simulink model "PMSM_SMO_Luenberger"  (R2024b)
settings: Solver=FixedStepDiscrete  StartTime=0.0  StopTime=2.4  FixedStep=TsPlant  RelTol=1e-3
InitFcn:
  | demoModel=bdroot; demoWorkspace=get_param(demoModel,'ModelWorkspace');
  | demoCases=getVariable(demoWorkspace,'DemoCases');
  | demoCaseName=get_param([demoModel '/Experiment_Settings'],'CaseName');
  | demoSelected=find(strcmp(demoCaseName,{demoCases.name}),1);
  | demoValues=demoCases(demoSelected).variables; demoNames=fieldnames(demoValues);
  | for demoIndex=1:numel(demoNames), assignin(demoWorkspace,demoNames{demoIndex},demoValues.(demoNames{demoIndex})); end
  | clear demoModel demoWorkspace demoCases demoCaseName demoSelected demoValues demoNames demoIndex;
model workspace (MAT data in the model file):
  CurrentKi = 720
  CurrentKp = 5.4
  DemoCases : object (value not decoded)
  EFilterA = 0.950976923294
  EFilterHz = 160
  FluxPM = 0.045
  FrictionB = 0.0001
  InertiaJ = 0.00025
  LsActual = 0.003
  LsNom = 0.003
  LuenL1 = 528.165269456
  LuenL2 = 575.388341705
  LuenPLLKi = 394784.176044
  LuenPLLKp = 1095.31763963
  PLLKi = 15791.3670417
  PLLKp = 177.688480487
  PWMfreq = 20000
  PolePairs = 4
  RsActual = 0.4
  RsNom = 0.4
  SmoK = 17.2906443411
  SmoKe = 0.821531981197
  SmoM = 33333.3333333
  SmoPLLKi = 116919.038546
  SmoPLLKp = 483.495044434
  SmoPhi = 0.315914362573
  SmoWmin = 100
  SpeedFilterA = 0.987512256524
  SpeedKi = 0.4
  SpeedKp = 0.04
  ThetaInitial = 0
  TsControl = 5e-05
  TsPlant = 2.5e-06
  TsSpeed = 0.001
  Vdc = 48
  inverterMode = 0
  loadStep = 0.18
  noiseTsABC = timeseries
  noiseTsABC.Name = 'unnamed'
  noiseTsABC.DataInfo = tsdata.datametadata
  noiseTsABC.DataInfo.Interpolation = tsdata.interpolation
  noiseTsABC.DataInfo.Interpolation.Fhandle : function handle (value not decoded)
  noiseTsABC.DataInfo.Interpolation.Name = 'linear'
  noiseTsABC.TimeInfo = tsdata.timemetadata
  noiseTsABC.TimeInfo.Length = 48001
  noiseTsABC.TimeInfo.DuplicateTimes = 0
  noiseTsABC.TimeInfo.Time_ = [0 5e-05 0.0001 0.00015 0.0002 0.00025 0.0003 0.00035 0.0004 0.00045 0.0005 0.00055 ... (48001 elements, 48001x1)]
  noiseTsABC.TimeInfo.Initialized = 1
  noiseTsABC.QualityInfo = tsdata.qualmetadata
  noiseTsABC.Data_ = [-0.0189584791563 -0.0055660672953 -0.00857497820907 -0.0128644236526 0.0199755803207 -0.0011001642805 0.0163280309249 -0.016225075147 0.00870875726314 -0.0018724684667 0.00550338350148 -0.000938030229996 ... (144003 elements, 48001x3)]
  rpm0 = 700
  rpm1 = 1000
  voltageErrorTs = timeseries
  voltageErrorTs.Name = 'unnamed'
  voltageErrorTs.DataInfo = tsdata.datametadata
  voltageErrorTs.DataInfo.Interpolation = tsdata.interpolation
  voltageErrorTs.DataInfo.Interpolation.Fhandle : function handle (value not decoded)
  voltageErrorTs.DataInfo.Interpolation.Name = 'linear'
  voltageErrorTs.TimeInfo = tsdata.timemetadata
  voltageErrorTs.TimeInfo.Length = 48001
  voltageErrorTs.TimeInfo.DuplicateTimes = 0
  voltageErrorTs.TimeInfo.Time_ = [0 5e-05 0.0001 0.00015 0.0002 0.00025 0.0003 0.00035 0.0004 0.00045 0.0005 0.00055 ... (48001 elements, 48001x1)]
  voltageErrorTs.TimeInfo.Initialized = 1
  voltageErrorTs.QualityInfo = tsdata.qualmetadata
  voltageErrorTs.Data_ = [0 0 0 0 0 0 0 0 0 0 0 0 ... (96002 elements, 48001x2)]
undefined symbols (not defined in the file): DiscIntNeverNeededParam
settings Model: Creator=lxy  LastModifiedBy=lxy

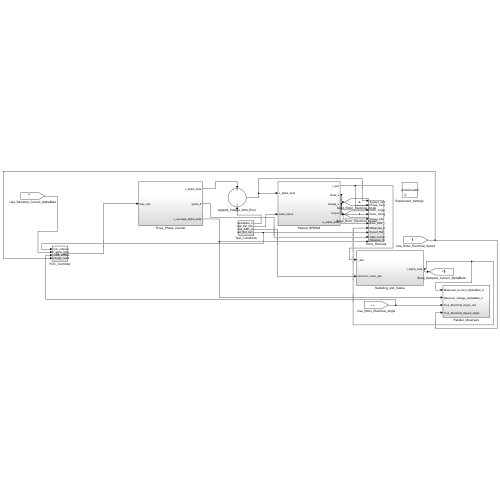
[thumbnail: Simulink's stored preview of the top-level diagram]
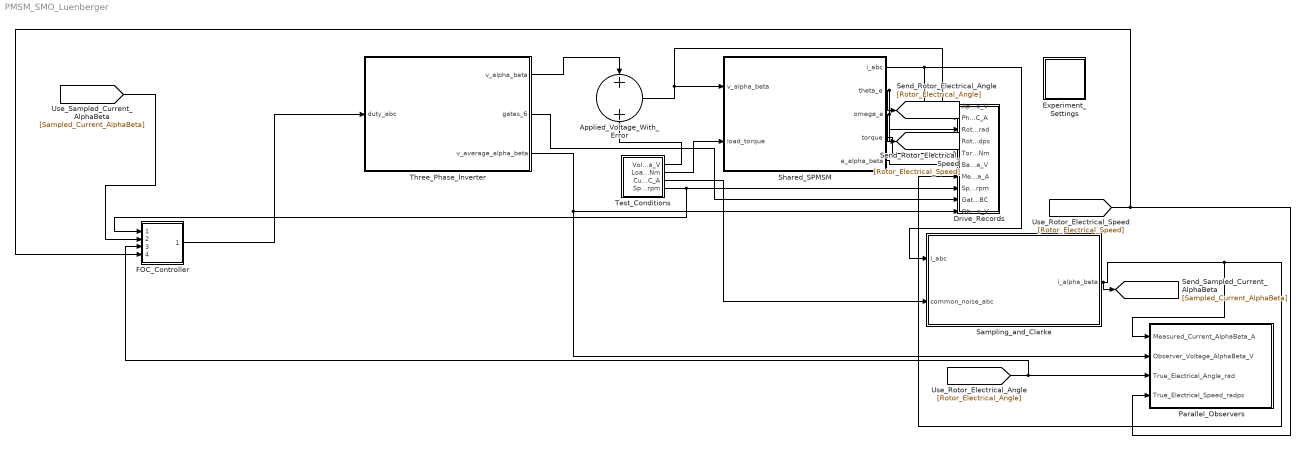
== system PMSM_SMO_Luenberger ==
  Applied_Voltage_With_Error : Sum
  Drive_Records : Subsystem
  Experiment_Settings : Subsystem  mask{CaseName=nominal}
      mask prompts: CaseName "Experiment"
      mask help: Select the experiment, then click Run. Parameters and test inputs are included in the download.
      mask TypeOptions CaseName: nominal | noise | mismatch | low_speed | zero_speed | ccf_narrow | ccf_wide | switched | voltage_bias | current_impulse | warm_resistance | heavy_load
      mask Display: disp('Experiment settings')
  FOC_Controller : Subsystem
  Parallel_Observers : Subsystem
  Sampling_and_Clarke : Subsystem
  Shared_SPMSM : Subsystem
  Test_Conditions : Subsystem
  Three_Phase_Inverter : Subsystem
  wires:
  Three_Phase_Inverter/1(v_alpha_beta) -> Applied_Voltage_With_Error/1
  Test_Conditions/3(Current_Noise_ABC_A) -> Sampling_and_Clarke/2(common_noise_abc)
  Test_Conditions/2(Load_Ref_Nm) -> Shared_SPMSM/2(load_torque)
  Test_Conditions/1(Voltage_Offset_AlphaBeta_V) -> Applied_Voltage_With_Error/2
  Shared_SPMSM/2(theta_e) -> [Rotor_Electrical_Angle], Drive_Records/3(Rotor_Angle_rad)
  Shared_SPMSM/1(i_abc) -> Sampling_and_Clarke/1(i_abc), Drive_Records/2(Phase_Current_ABC_A)
  Applied_Voltage_With_Error/1 -> Shared_SPMSM/1(v_alpha_beta), Drive_Records/1(Applied_Voltage_AlphaBeta_V)
  Shared_SPMSM/4(torque) -> Drive_Records/5(Torque_Nm)
  Shared_SPMSM/5(e_alpha_beta) -> Drive_Records/6(Back_EMF_AlphaBeta_V)
  Three_Phase_Inverter/2(gates_6) -> Drive_Records/9(Gate_Commands_ABC)
  [Sampled_Current_AlphaBeta] -> FOC_Controller/2(i_alpha_beta)
  Shared_SPMSM/3(omega_e) -> [Rotor_Electrical_Speed], Drive_Records/4(Rotor_Omega_radps)
  Test_Conditions/4(Speed_Ref_rpm) -> Drive_Records/8(Speed_Ref_rpm), FOC_Controller/1(rpm_reference)
  FOC_Controller/1(duty_abc) -> Three_Phase_Inverter/1(duty_abc)
  [Rotor_Electrical_Angle] -> Parallel_Observers/3(True_Electrical_Angle_rad), FOC_Controller/3(theta_feedback)
  [Rotor_Electrical_Speed] -> Parallel_Observers/4(True_Electrical_Speed_radps), FOC_Controller/4(omega_feedback)
  Three_Phase_Inverter/3(v_average_alpha_beta) -> Drive_Records/10(Observer_Voltage_AlphaBeta_V), Parallel_Observers/2(Observer_Voltage_AlphaBeta_V)
  Sampling_and_Clarke/1(i_alpha_beta) -> Parallel_Observers/1(Measured_Current_AlphaBeta_A), Drive_Records/7(Measured_Current_AlphaBeta_A), [Sampled_Current_AlphaBeta]

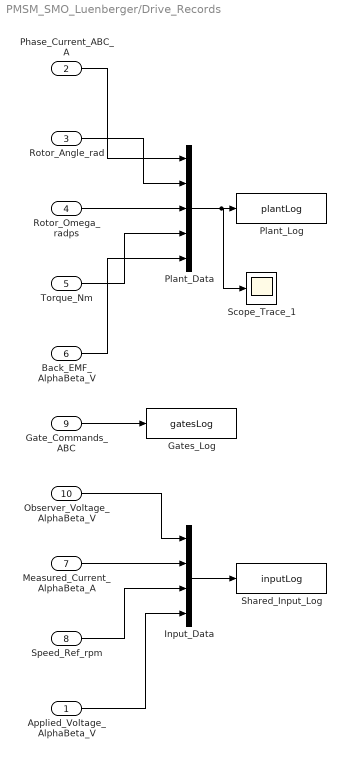
== system PMSM_SMO_Luenberger/Drive_Records ==
  Applied_Voltage_AlphaBeta_V : Inport
  Phase_Current_ABC_A : Inport  Port=2
  Rotor_Angle_rad : Inport  Port=3
  Rotor_Omega_radps : Inport  Port=4
  Torque_Nm : Inport  Port=5
  Back_EMF_AlphaBeta_V : Inport  Port=6
  Measured_Current_AlphaBeta_A : Inport  Port=7
  Speed_Ref_rpm : Inport  Port=8
  Gate_Commands_ABC : Inport  Port=9
  Observer_Voltage_AlphaBeta_V : Inport  Port=10
  Gates_Log : ToWorkspace  VariableName=gatesLog  SaveFormat=Timeseries
  Input_Data : Mux
  Plant_Data : Mux  Inputs=5
  Plant_Log : ToWorkspace  VariableName=plantLog  SaveFormat=Timeseries
  Scope_Trace_1 : Scope
  Shared_Input_Log : ToWorkspace  VariableName=inputLog  SaveFormat=Timeseries
  wires:
  Applied_Voltage_AlphaBeta_V/1 -> Input_Data/4
  Speed_Ref_rpm/1 -> Input_Data/3
  Measured_Current_AlphaBeta_A/1 -> Input_Data/2
  Observer_Voltage_AlphaBeta_V/1 -> Input_Data/1
  Rotor_Omega_radps/1 -> Plant_Data/3
  Back_EMF_AlphaBeta_V/1 -> Plant_Data/5
  Gate_Commands_ABC/1 -> Gates_Log/1
  Torque_Nm/1 -> Plant_Data/4
  Rotor_Angle_rad/1 -> Plant_Data/2
  Phase_Current_ABC_A/1 -> Plant_Data/1
  Input_Data/1 -> Shared_Input_Log/1
  Plant_Data/1 -> Scope_Trace_1/1, Plant_Log/1

== system PMSM_SMO_Luenberger/Experiment_Settings ==

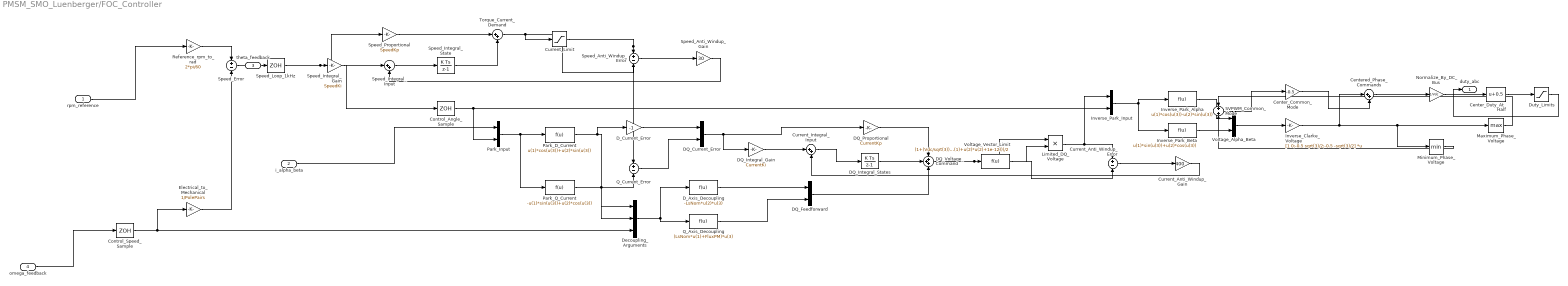
== system PMSM_SMO_Luenberger/FOC_Controller ==
  rpm_reference : Inport
  i_alpha_beta : Inport  Port=2
  theta_feedback : Inport  Port=3
  omega_feedback : Inport  Port=4
  Center_Common_Mode : Gain  Gain=-0.5
  Center_Duty_At_Half : Bias  Bias=0.5
  Centered_Phase_Commands : Sum  Inputs=|++
  Control_Angle_Sample : ZeroOrderHold  SampleTime=TsControl
  Control_Speed_Sample : ZeroOrderHold  SampleTime=TsControl
  Current_Anti_Windup_Error : Sum  Inputs=+-
  Current_Anti_Windup_Gain : Gain  Gain=400
  Current_Integral_Input : Sum  Inputs=|++
  Current_Limit : Saturate  UpperLimit=4  LowerLimit=-4
  DQ_Current_Error : Mux  Inputs=2
  DQ_Feedforward : Mux  Inputs=2
  DQ_Integral_Gain : Gain  Gain=CurrentKi
  DQ_Integral_States : DiscreteIntegrator  InitialCondition=[0;0]  SampleTime=TsControl  ICPrevOutput=DiscIntNeverNeededParam  ICPrevScaledInput=DiscIntNeverNeededParam
  DQ_Proportional : Gain  Gain=CurrentKp
  DQ_Voltage_Command : Sum  Inputs=+++
  D_Axis_Decoupling : Fcn  Expr=-LsNom*u(2)*u(3)
  D_Current_Error : Gain  Gain=-1
  Decoupling_Arguments : Mux  Inputs=3
  Duty_Limits : Saturate  UpperLimit=1  LowerLimit=0
  Electrical_to_Mechanical : Gain  Gain=1/PolePairs
  Inverse_Clarke_Voltage : Gain  Gain=[1 0;-0.5 sqrt(3)/2;-0.5 -sqrt(3)/2]  Multiplication=Matrix(K*u)
  Inverse_Park_Alpha : Fcn  Expr=u(1)*cos(u(3))-u(2)*sin(u(3))
  Inverse_Park_Beta : Fcn  Expr=u(1)*sin(u(3))+u(2)*cos(u(3))
  Inverse_Park_Input : Mux  Inputs=2
  Limited_DQ_Voltage : Product  Inputs=**
  Maximum_Phase_Voltage : MinMax  Function=max
  Minimum_Phase_Voltage : MinMax
  Normalize_By_DC_Bus : Gain  Gain=1/Vdc
  Park_D_Current : Fcn  Expr=u(1)*cos(u(3))+u(2)*sin(u(3))
  Park_Input : Mux  Inputs=2
  Park_Q_Current : Fcn  Expr=-u(1)*sin(u(3))+u(2)*cos(u(3))
  Q_Axis_Decoupling : Fcn  Expr=(LsNom*u(1)+FluxPM)*u(3)
  Q_Current_Error : Sum  Inputs=+-
  Reference_rpm_to_rad : Gain  Gain=2*pi/60
  SVPWM_Common_Mode : Sum
  Speed_Anti_Windup_Error : Sum  Inputs=+-
  Speed_Anti_Windup_Gain : Gain  Gain=30
  Speed_Error : Sum  Inputs=+-
  Speed_Integral_Gain : Gain  Gain=SpeedKi
  Speed_Integral_Input : Sum  Inputs=|++
  Speed_Integral_State : DiscreteIntegrator  SampleTime=TsSpeed  ICPrevOutput=DiscIntNeverNeededParam  ICPrevScaledInput=DiscIntNeverNeededParam
  Speed_Loop_1kHz : ZeroOrderHold  SampleTime=TsSpeed
  Speed_Proportional : Gain  Gain=SpeedKp
  Torque_Current_Demand : Sum  Inputs=|++
  Voltage_Alpha_Beta : Mux  Inputs=2
  Voltage_Vector_Limit : Fcn  Expr=(1+(Vdc/sqrt(3))/sqrt(u(1)*u(1)+u(2)*u(2)+1e-12)-abs(1-(Vdc/sqrt(3))/sqrt(u(1)*u(1)+u(2)*u(2)+1e-12)))/2
  duty_abc : Outport
  wires:
  Duty_Limits/1 -> duty_abc/1
  Center_Duty_At_Half/1 -> Duty_Limits/1
  Normalize_By_DC_Bus/1 -> Center_Duty_At_Half/1
  Centered_Phase_Commands/1 -> Normalize_By_DC_Bus/1
  Inverse_Clarke_Voltage/1 -> Maximum_Phase_Voltage/1, Minimum_Phase_Voltage/1, Centered_Phase_Commands/1
  Voltage_Alpha_Beta/1 -> Inverse_Clarke_Voltage/1
  Inverse_Park_Beta/1 -> Voltage_Alpha_Beta/2
  Inverse_Park_Alpha/1 -> Voltage_Alpha_Beta/1
  Inverse_Park_Input/1 -> Inverse_Park_Beta/1, Inverse_Park_Alpha/1
  Current_Integral_Input/1 -> DQ_Integral_States/1
  Current_Anti_Windup_Gain/1 -> Current_Integral_Input/2
  DQ_Integral_Gain/1 -> Current_Integral_Input/1
  Current_Anti_Windup_Error/1 -> Current_Anti_Windup_Gain/1
  Limited_DQ_Voltage/1 -> Inverse_Park_Input/1, Current_Anti_Windup_Error/1
  Voltage_Vector_Limit/1 -> Limited_DQ_Voltage/2
  DQ_Voltage_Command/1 -> Limited_DQ_Voltage/1, Current_Anti_Windup_Error/2, Voltage_Vector_Limit/1
  DQ_Feedforward/1 -> DQ_Voltage_Command/3
  Q_Axis_Decoupling/1 -> DQ_Feedforward/2
  D_Axis_Decoupling/1 -> DQ_Feedforward/1
  Decoupling_Arguments/1 -> D_Axis_Decoupling/1, Q_Axis_Decoupling/1
  DQ_Integral_States/1 -> DQ_Voltage_Command/2
  DQ_Proportional/1 -> DQ_Voltage_Command/1
  DQ_Current_Error/1 -> DQ_Integral_Gain/1, DQ_Proportional/1
  Q_Current_Error/1 -> DQ_Current_Error/2
  D_Current_Error/1 -> DQ_Current_Error/1
  Park_Q_Current/1 -> Decoupling_Arguments/2, Q_Current_Error/2
  Park_D_Current/1 -> D_Current_Error/1, Decoupling_Arguments/1
  Park_Input/1 -> Park_Q_Current/1, Park_D_Current/1
  Control_Angle_Sample/1 -> Park_Input/2, Inverse_Park_Input/2
  i_alpha_beta/1 -> Park_Input/1
  Speed_Integral_Input/1 -> Speed_Integral_State/1
  Speed_Anti_Windup_Gain/1 -> Speed_Integral_Input/2
  Speed_Integral_Gain/1 -> Speed_Integral_Input/1
  Speed_Anti_Windup_Error/1 -> Speed_Anti_Windup_Gain/1
  Current_Limit/1 -> Speed_Anti_Windup_Error/1, Q_Current_Error/1
  Torque_Current_Demand/1 -> Current_Limit/1, Speed_Anti_Windup_Error/2
  Speed_Integral_State/1 -> Torque_Current_Demand/2
  Speed_Proportional/1 -> Torque_Current_Demand/1
  Speed_Loop_1kHz/1 -> Speed_Integral_Gain/1, Speed_Proportional/1
  Speed_Error/1 -> Speed_Loop_1kHz/1
  Electrical_to_Mechanical/1 -> Speed_Error/2
  Reference_rpm_to_rad/1 -> Speed_Error/1
  Control_Speed_Sample/1 -> Electrical_to_Mechanical/1, Decoupling_Arguments/3
  rpm_reference/1 -> Reference_rpm_to_rad/1
  omega_feedback/1 -> Control_Speed_Sample/1
  theta_feedback/1 -> Control_Angle_Sample/1
  Center_Common_Mode/1 -> Centered_Phase_Commands/2
  Maximum_Phase_Voltage/1 -> SVPWM_Common_Mode/1
  Minimum_Phase_Voltage/1 -> SVPWM_Common_Mode/2
  SVPWM_Common_Mode/1 -> Center_Common_Mode/1

== system PMSM_SMO_Luenberger/Parallel_Observers ==
  Measured_Current_AlphaBeta_A : Inport
  Observer_Voltage_AlphaBeta_V : Inport  Port=2
  True_Electrical_Angle_rad : Inport  Port=3
  True_Electrical_Speed_radps : Inport  Port=4
  Luenberger : Subsystem
  Luenberger_Angle_Speed : Demux  Outputs=2
  Luenberger_Data : Mux
  Luenberger_Log : ToWorkspace  VariableName=luenLog  SaveFormat=Timeseries
  SMO : Subsystem
  SMO_Angle_Speed : Demux  Outputs=2
  SMO_Data : Mux
  SMO_Log : ToWorkspace  VariableName=smoLog  SaveFormat=Timeseries
  Scope_Angle_rad : Scope  NumInputPorts=3
  Scope_Electrical_Speed_radps : Scope  NumInputPorts=3
  wires:
  Luenberger/4(correction_V) -> Luenberger_Data/4
  SMO/2(omega_e) -> SMO_Data/2
  Luenberger/2(omega_e) -> Luenberger_Data/2
  Luenberger/3(e_alpha_beta) -> Luenberger_Data/3
  Luenberger/1(theta_e) -> Luenberger_Data/1
  SMO/1(theta_e) -> SMO_Data/1
  SMO/4(correction_V) -> SMO_Data/4
  SMO/3(e_alpha_beta) -> SMO_Data/3
  Observer_Voltage_AlphaBeta_V/1 -> Luenberger/1(v_alpha_beta), SMO/1(v_alpha_beta)
  Measured_Current_AlphaBeta_A/1 -> SMO/2(i_alpha_beta), Luenberger/2(i_alpha_beta)
  SMO_Angle_Speed/2 -> Scope_Electrical_Speed_radps/3
  Luenberger_Angle_Speed/2 -> Scope_Electrical_Speed_radps/2
  True_Electrical_Speed_radps/1 -> Scope_Electrical_Speed_radps/1
  SMO_Angle_Speed/1 -> Scope_Angle_rad/3
  Luenberger_Angle_Speed/1 -> Scope_Angle_rad/2
  True_Electrical_Angle_rad/1 -> Scope_Angle_rad/1
  SMO_Data/1 -> SMO_Angle_Speed/1, SMO_Log/1
  Luenberger_Data/1 -> Luenberger_Angle_Speed/1, Luenberger_Log/1

== system PMSM_SMO_Luenberger/Sampling_and_Clarke ==
  i_abc : Inport
  common_noise_abc : Inport  Port=2
  ADC_Sample_and_Hold : ZeroOrderHold  SampleTime=TsControl
  Add_Common_ADC_Noise : Sum  Inputs=|++
  Clarke_Transformation : Gain  Gain=[2/3 -1/3 -1/3;0 1/sqrt(3) -1/sqrt(3)]  Multiplication=Matrix(K*u)
  i_alpha_beta : Outport
  wires:
  Clarke_Transformation/1 -> i_alpha_beta/1
  ADC_Sample_and_Hold/1 -> Clarke_Transformation/1
  Add_Common_ADC_Noise/1 -> ADC_Sample_and_Hold/1
  common_noise_abc/1 -> Add_Common_ADC_Noise/2
  i_abc/1 -> Add_Common_ADC_Noise/1

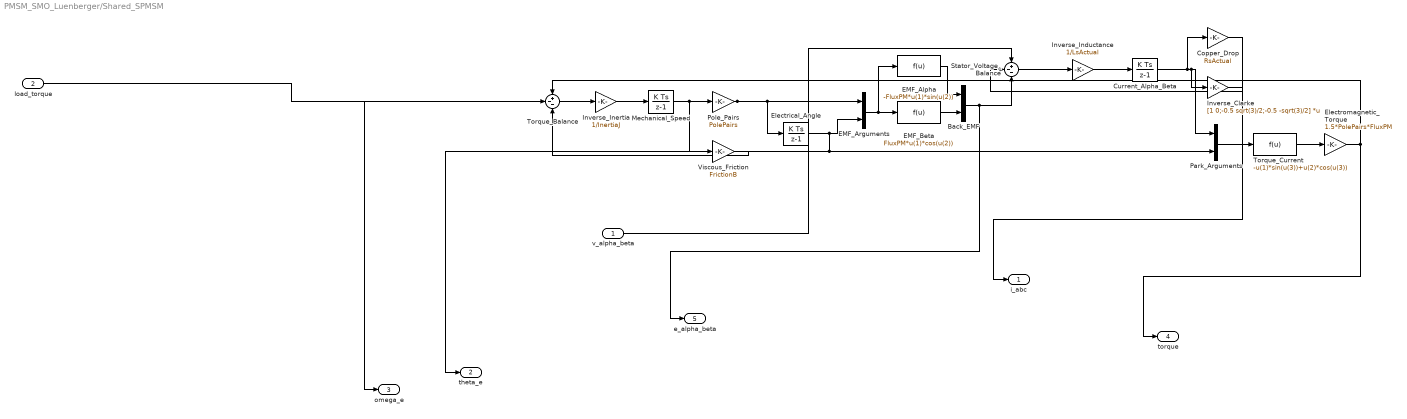
== system PMSM_SMO_Luenberger/Shared_SPMSM ==
  v_alpha_beta : Inport
  load_torque : Inport  Port=2
  Back_EMF : Mux  Inputs=2
  Copper_Drop : Gain  Gain=RsActual
  Current_Alpha_Beta : DiscreteIntegrator  InitialCondition=[0;0]  SampleTime=TsPlant  ICPrevOutput=DiscIntNeverNeededParam  ICPrevScaledInput=DiscIntNeverNeededParam
  EMF_Alpha : Fcn  Expr=-FluxPM*u(1)*sin(u(2))
  EMF_Arguments : Mux  Inputs=2
  EMF_Beta : Fcn  Expr=FluxPM*u(1)*cos(u(2))
  Electrical_Angle : DiscreteIntegrator  InitialCondition=ThetaInitial  SampleTime=TsPlant  ICPrevOutput=DiscIntNeverNeededParam  ICPrevScaledInput=DiscIntNeverNeededParam
  Electromagnetic_Torque : Gain  Gain=1.5*PolePairs*FluxPM
  Inverse_Clarke : Gain  Gain=[1 0;-0.5 sqrt(3)/2;-0.5 -sqrt(3)/2]  Multiplication=Matrix(K*u)
  Inverse_Inductance : Gain  Gain=1/LsActual
  Inverse_Inertia : Gain  Gain=1/InertiaJ
  Mechanical_Speed : DiscreteIntegrator  SampleTime=TsPlant  ICPrevOutput=DiscIntNeverNeededParam  ICPrevScaledInput=DiscIntNeverNeededParam
  Park_Arguments : Mux  Inputs=2
  Pole_Pairs : Gain  Gain=PolePairs
  Stator_Voltage_Balance : Sum  Inputs=+--
  Torque_Balance : Sum  Inputs=+--
  Torque_Current : Fcn  Expr=-u(1)*sin(u(3))+u(2)*cos(u(3))
  Viscous_Friction : Gain  Gain=FrictionB
  i_abc : Outport
  theta_e : Outport  Port=2
  omega_e : Outport  Port=3
  torque : Outport  Port=4
  e_alpha_beta : Outport  Port=5
  wires:
  Inverse_Inertia/1 -> Mechanical_Speed/1
  Torque_Balance/1 -> Inverse_Inertia/1
  Viscous_Friction/1 -> Torque_Balance/3
  load_torque/1 -> Torque_Balance/2
  Electromagnetic_Torque/1 -> Torque_Balance/1, torque/1
  Torque_Current/1 -> Electromagnetic_Torque/1
  Park_Arguments/1 -> Torque_Current/1
  EMF_Beta/1 -> Back_EMF/2
  EMF_Alpha/1 -> Back_EMF/1
  EMF_Arguments/1 -> EMF_Alpha/1, EMF_Beta/1
  Electrical_Angle/1 -> Park_Arguments/2, theta_e/1, EMF_Arguments/2
  Pole_Pairs/1 -> EMF_Arguments/1, Electrical_Angle/1, omega_e/1
  Mechanical_Speed/1 -> Pole_Pairs/1, Viscous_Friction/1
  Inverse_Clarke/1 -> i_abc/1
  Inverse_Inductance/1 -> Current_Alpha_Beta/1
  Stator_Voltage_Balance/1 -> Inverse_Inductance/1
  Back_EMF/1 -> e_alpha_beta/1, Stator_Voltage_Balance/3
  Copper_Drop/1 -> Stator_Voltage_Balance/2
  Current_Alpha_Beta/1 -> Copper_Drop/1, Park_Arguments/1, Inverse_Clarke/1
  v_alpha_beta/1 -> Stator_Voltage_Balance/1

== system PMSM_SMO_Luenberger/Test_Conditions ==
  Applied_Voltage_Error : FromWorkspace  VariableName=voltageErrorTs  Interpolate=off  OutputAfterFinalValue=Holding final value
  Common_Sensor_Noise : FromWorkspace  VariableName=noiseTsABC
  Load_Torque_Nm : Step  Time=1.6  After=loadStep  SampleTime=TsPlant
  Speed_Reference_rpm : Step  Before=rpm0  After=rpm1  SampleTime=TsControl
  Voltage_Offset_AlphaBeta_V : Outport
  Load_Ref_Nm : Outport  Port=2
  Current_Noise_ABC_A : Outport  Port=3
  Speed_Ref_rpm : Outport  Port=4
  wires:
  Load_Torque_Nm/1 -> Load_Ref_Nm/1
  Applied_Voltage_Error/1 -> Voltage_Offset_AlphaBeta_V/1
  Common_Sensor_Noise/1 -> Current_Noise_ABC_A/1
  Speed_Reference_rpm/1 -> Speed_Ref_rpm/1

== system PMSM_SMO_Luenberger/Three_Phase_Inverter ==
  duty_abc : Inport
  Average_Voltage_Clarke : Gain  Gain=[2/3 -1/3 -1/3;0 1/sqrt(3) -1/sqrt(3)]  Multiplication=Matrix(K*u)
  Average_or_Switched : Switch  Threshold=0.5
  Carrier_Time : Clock
  Center_Aligned_Carrier : Fcn  Expr=abs(2*(u*PWMfreq-floor(u*PWMfreq))-1)
  Complementary_Lower_Gates : Logic  Operator=NOT  IconShape=distinctive
  DC_Bus_Average_Poles : Gain  Gain=Vdc
  DC_Bus_Switched_Poles : Gain  Gain=Vdc  OutDataTypeStr=double
  Inverter_Mode : Constant  Value=inverterMode
  Pole_to_Alpha_Beta : Gain  Gain=[2/3 -1/3 -1/3;0 1/sqrt(3) -1/sqrt(3)]  Multiplication=Matrix(K*u)
  Six_Gate_Signals : Mux  Inputs=2
  Upper_Bridge_Gates : RelationalOperator  Operator=>
  v_alpha_beta : Outport
  gates_6 : Outport  Port=2
  v_average_alpha_beta : Outport  Port=3
  wires:
  Average_Voltage_Clarke/1 -> v_average_alpha_beta/1
  Pole_to_Alpha_Beta/1 -> v_alpha_beta/1
  Average_or_Switched/1 -> Pole_to_Alpha_Beta/1
  DC_Bus_Average_Poles/1 -> Average_Voltage_Clarke/1, Average_or_Switched/3
  Inverter_Mode/1 -> Average_or_Switched/2
  DC_Bus_Switched_Poles/1 -> Average_or_Switched/1
  Six_Gate_Signals/1 -> gates_6/1
  Complementary_Lower_Gates/1 -> Six_Gate_Signals/2
  Upper_Bridge_Gates/1 -> Six_Gate_Signals/1, Complementary_Lower_Gates/1, DC_Bus_Switched_Poles/1
  Center_Aligned_Carrier/1 -> Upper_Bridge_Gates/2
  Carrier_Time/1 -> Center_Aligned_Carrier/1
  duty_abc/1 -> Upper_Bridge_Gates/1, DC_Bus_Average_Poles/1

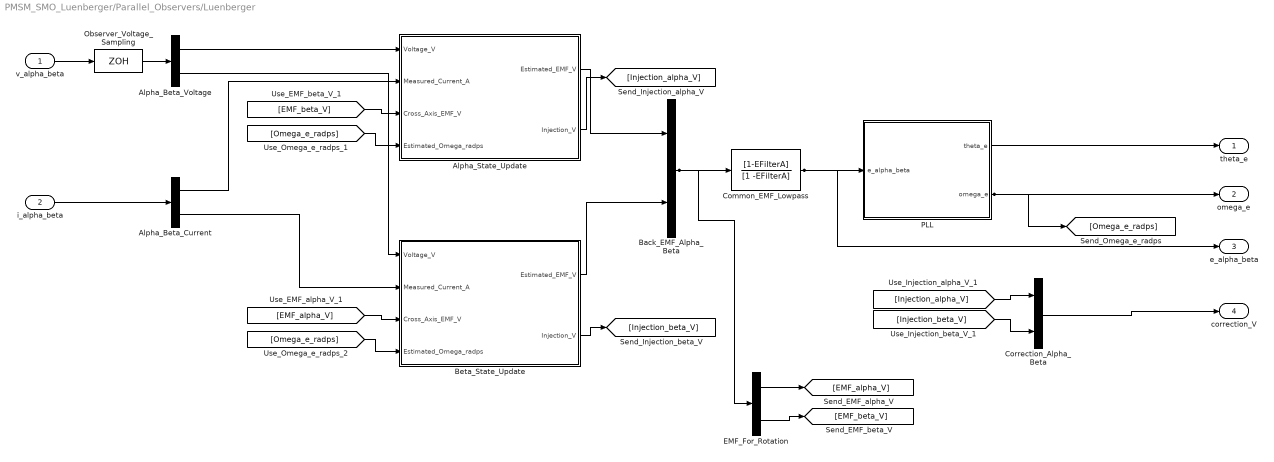
== system PMSM_SMO_Luenberger/Parallel_Observers/Luenberger ==
  v_alpha_beta : Inport
  i_alpha_beta : Inport  Port=2
  Alpha_Beta_Current : Demux  Outputs=2
  Alpha_Beta_Voltage : Demux  Outputs=2
  Alpha_State_Update : Subsystem
  Back_EMF_Alpha_Beta : Mux  Inputs=2
  Beta_State_Update : Subsystem
  Common_EMF_Lowpass : DiscreteTransferFcn  Numerator=[1-EFilterA]  Denominator=[1 -EFilterA]  SampleTime=TsControl
  Correction_Alpha_Beta : Mux  Inputs=2
  EMF_For_Rotation : Demux  Outputs=2
  Observer_Voltage_Sampling : ZeroOrderHold  SampleTime=TsControl
  PLL : Subsystem
  theta_e : Outport
  omega_e : Outport  Port=2
  e_alpha_beta : Outport  Port=3
  correction_V : Outport  Port=4
  wires:
  Beta_State_Update/1(Estimated_EMF_V) -> Back_EMF_Alpha_Beta/2
  Alpha_Beta_Current/2 -> Beta_State_Update/2(Measured_Current_A)
  Alpha_Beta_Voltage/2 -> Beta_State_Update/1(Voltage_V)
  Alpha_State_Update/1(Estimated_EMF_V) -> Back_EMF_Alpha_Beta/1
  Alpha_Beta_Current/1 -> Alpha_State_Update/2(Measured_Current_A)
  Alpha_Beta_Voltage/1 -> Alpha_State_Update/1(Voltage_V)
  v_alpha_beta/1 -> Observer_Voltage_Sampling/1
  Observer_Voltage_Sampling/1 -> Alpha_Beta_Voltage/1
  i_alpha_beta/1 -> Alpha_Beta_Current/1
  Back_EMF_Alpha_Beta/1 -> EMF_For_Rotation/1, Common_EMF_Lowpass/1
  Common_EMF_Lowpass/1 -> e_alpha_beta/1, PLL/1(e_alpha_beta)
  PLL/1(theta_e) -> theta_e/1
  Correction_Alpha_Beta/1 -> correction_V/1
  [EMF_alpha_V] -> Beta_State_Update/3(Cross_Axis_EMF_V)
  EMF_For_Rotation/1 -> [EMF_alpha_V]
  [EMF_beta_V] -> Alpha_State_Update/3(Cross_Axis_EMF_V)
  EMF_For_Rotation/2 -> [EMF_beta_V]
  [Omega_e_radps] -> Beta_State_Update/4(Estimated_Omega_radps)
  [Omega_e_radps] -> Alpha_State_Update/4(Estimated_Omega_radps)
  PLL/2(omega_e) -> [Omega_e_radps], omega_e/1
  [Injection_alpha_V] -> Correction_Alpha_Beta/1
  Alpha_State_Update/2(Injection_V) -> [Injection_alpha_V]
  [Injection_beta_V] -> Correction_Alpha_Beta/2
  Beta_State_Update/2(Injection_V) -> [Injection_beta_V]

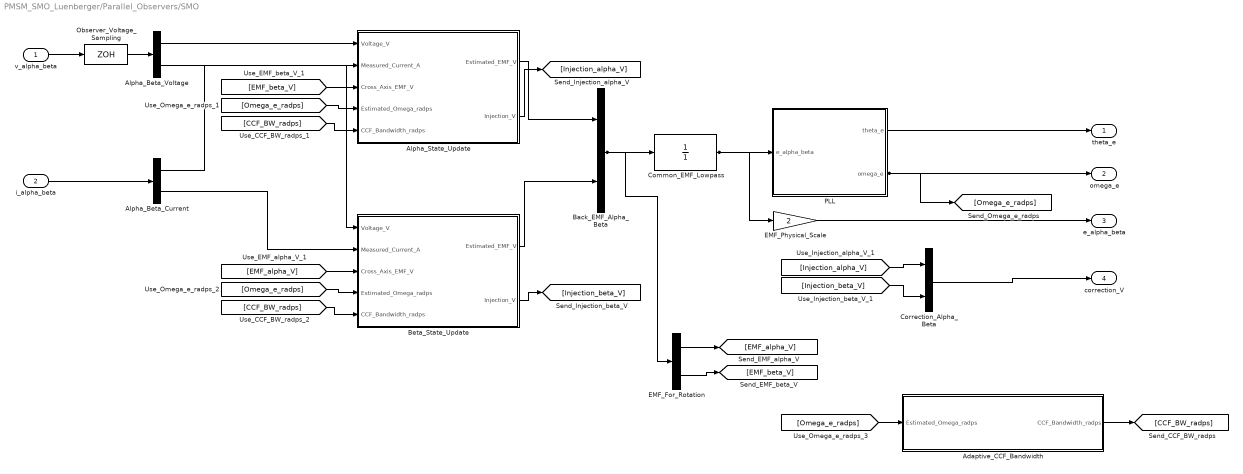
== system PMSM_SMO_Luenberger/Parallel_Observers/SMO ==
  v_alpha_beta : Inport
  i_alpha_beta : Inport  Port=2
  Adaptive_CCF_Bandwidth : Subsystem
  Alpha_Beta_Current : Demux  Outputs=2
  Alpha_Beta_Voltage : Demux  Outputs=2
  Alpha_State_Update : Subsystem
  Back_EMF_Alpha_Beta : Mux  Inputs=2
  Beta_State_Update : Subsystem
  Common_EMF_Lowpass : DiscreteTransferFcn  Denominator=[1]  SampleTime=TsControl
  Correction_Alpha_Beta : Mux  Inputs=2
  EMF_For_Rotation : Demux  Outputs=2
  EMF_Physical_Scale : Gain  Gain=2
  Observer_Voltage_Sampling : ZeroOrderHold  SampleTime=TsControl
  PLL : Subsystem
  theta_e : Outport
  omega_e : Outport  Port=2
  e_alpha_beta : Outport  Port=3
  correction_V : Outport  Port=4
  wires:
  Beta_State_Update/1(Estimated_EMF_V) -> Back_EMF_Alpha_Beta/2
  Alpha_Beta_Current/2 -> Beta_State_Update/2(Measured_Current_A)
  Alpha_Beta_Voltage/2 -> Beta_State_Update/1(Voltage_V)
  Alpha_State_Update/1(Estimated_EMF_V) -> Back_EMF_Alpha_Beta/1
  Alpha_Beta_Current/1 -> Alpha_State_Update/2(Measured_Current_A)
  Alpha_Beta_Voltage/1 -> Alpha_State_Update/1(Voltage_V)
  EMF_Physical_Scale/1 -> e_alpha_beta/1
  v_alpha_beta/1 -> Observer_Voltage_Sampling/1
  Observer_Voltage_Sampling/1 -> Alpha_Beta_Voltage/1
  i_alpha_beta/1 -> Alpha_Beta_Current/1
  Back_EMF_Alpha_Beta/1 -> Common_EMF_Lowpass/1, EMF_For_Rotation/1
  Common_EMF_Lowpass/1 -> EMF_Physical_Scale/1, PLL/1(e_alpha_beta)
  PLL/1(theta_e) -> theta_e/1
  Correction_Alpha_Beta/1 -> correction_V/1
  [EMF_alpha_V] -> Beta_State_Update/3(Cross_Axis_EMF_V)
  EMF_For_Rotation/1 -> [EMF_alpha_V]
  [EMF_beta_V] -> Alpha_State_Update/3(Cross_Axis_EMF_V)
  EMF_For_Rotation/2 -> [EMF_beta_V]
  [Omega_e_radps] -> Beta_State_Update/4(Estimated_Omega_radps)
  [Omega_e_radps] -> Alpha_State_Update/4(Estimated_Omega_radps)
  PLL/2(omega_e) -> omega_e/1, [Omega_e_radps]
  [CCF_BW_radps] -> Beta_State_Update/5(CCF_Bandwidth_radps)
  [CCF_BW_radps] -> Alpha_State_Update/5(CCF_Bandwidth_radps)
  Adaptive_CCF_Bandwidth/1(CCF_Bandwidth_radps) -> [CCF_BW_radps]
  [Omega_e_radps] -> Adaptive_CCF_Bandwidth/1(Estimated_Omega_radps)
  [Injection_alpha_V] -> Correction_Alpha_Beta/1
  Alpha_State_Update/2(Injection_V) -> [Injection_alpha_V]
  [Injection_beta_V] -> Correction_Alpha_Beta/2
  Beta_State_Update/2(Injection_V) -> [Injection_beta_V]

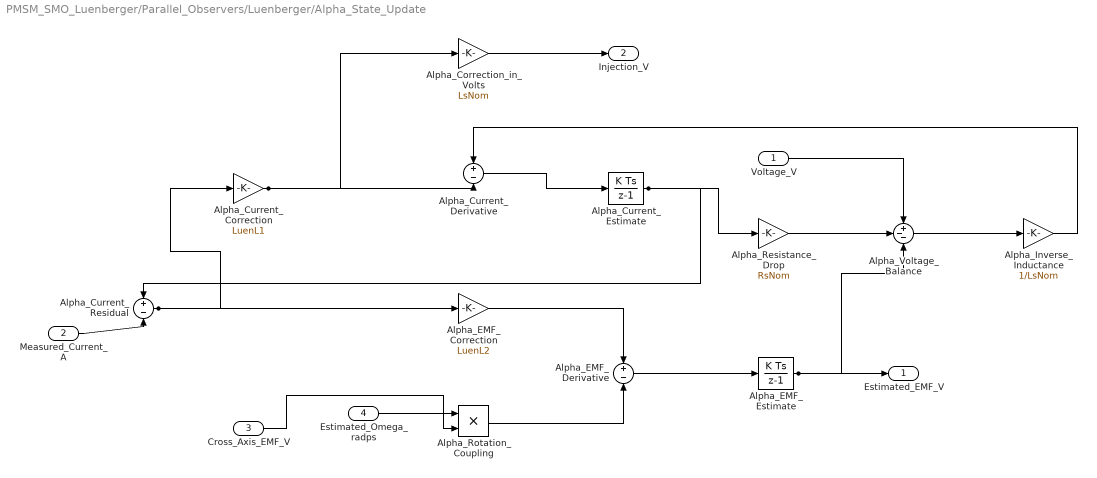
== system PMSM_SMO_Luenberger/Parallel_Observers/Luenberger/Alpha_State_Update ==
  Voltage_V : Inport
  Measured_Current_A : Inport  Port=2
  Cross_Axis_EMF_V : Inport  Port=3
  Estimated_Omega_radps : Inport  Port=4
  Alpha_Correction_in_Volts : Gain  Gain=LsNom
  Alpha_Current_Correction : Gain  Gain=LuenL1
  Alpha_Current_Derivative : Sum  Inputs=+-
  Alpha_Current_Estimate : DiscreteIntegrator  SampleTime=TsControl  ICPrevOutput=DiscIntNeverNeededParam  ICPrevScaledInput=DiscIntNeverNeededParam
  Alpha_Current_Residual : Sum  Inputs=+-
  Alpha_EMF_Correction : Gain  Gain=LuenL2
  Alpha_EMF_Derivative : Sum  Inputs=+-
  Alpha_EMF_Estimate : DiscreteIntegrator  SampleTime=TsControl  ICPrevOutput=DiscIntNeverNeededParam  ICPrevScaledInput=DiscIntNeverNeededParam
  Alpha_Inverse_Inductance : Gain  Gain=1/LsNom
  Alpha_Resistance_Drop : Gain  Gain=RsNom
  Alpha_Rotation_Coupling : Product  Inputs=**
  Alpha_Voltage_Balance : Sum  Inputs=+--
  Estimated_EMF_V : Outport
  Injection_V : Outport  Port=2
  wires:
  Alpha_EMF_Correction/1 -> Alpha_EMF_Derivative/1
  Alpha_EMF_Derivative/1 -> Alpha_EMF_Estimate/1
  Alpha_Resistance_Drop/1 -> Alpha_Voltage_Balance/2
  Alpha_Rotation_Coupling/1 -> Alpha_EMF_Derivative/2
  Alpha_Current_Residual/1 -> Alpha_Current_Correction/1, Alpha_EMF_Correction/1
  Alpha_Current_Correction/1 -> Alpha_Current_Derivative/2, Alpha_Correction_in_Volts/1
  Estimated_Omega_radps/1 -> Alpha_Rotation_Coupling/1
  Alpha_EMF_Estimate/1 -> Estimated_EMF_V/1, Alpha_Voltage_Balance/3
  Alpha_Voltage_Balance/1 -> Alpha_Inverse_Inductance/1
  Alpha_Inverse_Inductance/1 -> Alpha_Current_Derivative/1
  Alpha_Current_Estimate/1 -> Alpha_Resistance_Drop/1, Alpha_Current_Residual/1
  Cross_Axis_EMF_V/1 -> Alpha_Rotation_Coupling/2
  Alpha_Current_Derivative/1 -> Alpha_Current_Estimate/1
  Voltage_V/1 -> Alpha_Voltage_Balance/1
  Measured_Current_A/1 -> Alpha_Current_Residual/2
  Alpha_Correction_in_Volts/1 -> Injection_V/1

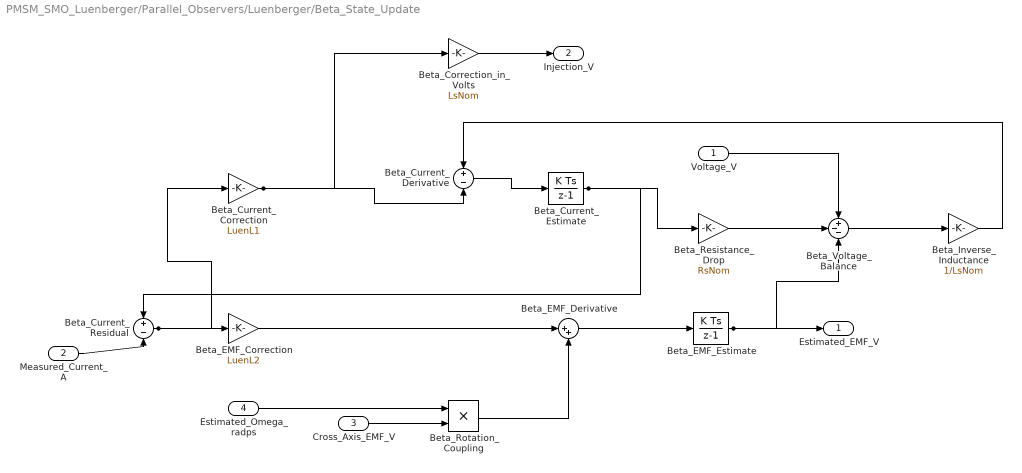
== system PMSM_SMO_Luenberger/Parallel_Observers/Luenberger/Beta_State_Update ==
  Voltage_V : Inport
  Measured_Current_A : Inport  Port=2
  Cross_Axis_EMF_V : Inport  Port=3
  Estimated_Omega_radps : Inport  Port=4
  Beta_Correction_in_Volts : Gain  Gain=LsNom
  Beta_Current_Correction : Gain  Gain=LuenL1
  Beta_Current_Derivative : Sum  Inputs=+-
  Beta_Current_Estimate : DiscreteIntegrator  SampleTime=TsControl  ICPrevOutput=DiscIntNeverNeededParam  ICPrevScaledInput=DiscIntNeverNeededParam
  Beta_Current_Residual : Sum  Inputs=+-
  Beta_EMF_Correction : Gain  Gain=LuenL2
  Beta_EMF_Derivative : Sum  Inputs=|++
  Beta_EMF_Estimate : DiscreteIntegrator  SampleTime=TsControl  ICPrevOutput=DiscIntNeverNeededParam  ICPrevScaledInput=DiscIntNeverNeededParam
  Beta_Inverse_Inductance : Gain  Gain=1/LsNom
  Beta_Resistance_Drop : Gain  Gain=RsNom
  Beta_Rotation_Coupling : Product  Inputs=**
  Beta_Voltage_Balance : Sum  Inputs=+--
  Estimated_EMF_V : Outport
  Injection_V : Outport  Port=2
  wires:
  Measured_Current_A/1 -> Beta_Current_Residual/2
  Voltage_V/1 -> Beta_Voltage_Balance/1
  Beta_Correction_in_Volts/1 -> Injection_V/1
  Beta_EMF_Derivative/1 -> Beta_EMF_Estimate/1
  Beta_Rotation_Coupling/1 -> Beta_EMF_Derivative/2
  Beta_EMF_Correction/1 -> Beta_EMF_Derivative/1
  Beta_Current_Residual/1 -> Beta_EMF_Correction/1, Beta_Current_Correction/1
  Beta_Current_Estimate/1 -> Beta_Current_Residual/1, Beta_Resistance_Drop/1
  Beta_Current_Derivative/1 -> Beta_Current_Estimate/1
  Estimated_Omega_radps/1 -> Beta_Rotation_Coupling/1
  Beta_EMF_Estimate/1 -> Beta_Voltage_Balance/3, Estimated_EMF_V/1
  Beta_Inverse_Inductance/1 -> Beta_Current_Derivative/1
  Beta_Resistance_Drop/1 -> Beta_Voltage_Balance/2
  Beta_Current_Correction/1 -> Beta_Correction_in_Volts/1, Beta_Current_Derivative/2
  Cross_Axis_EMF_V/1 -> Beta_Rotation_Coupling/2
  Beta_Voltage_Balance/1 -> Beta_Inverse_Inductance/1

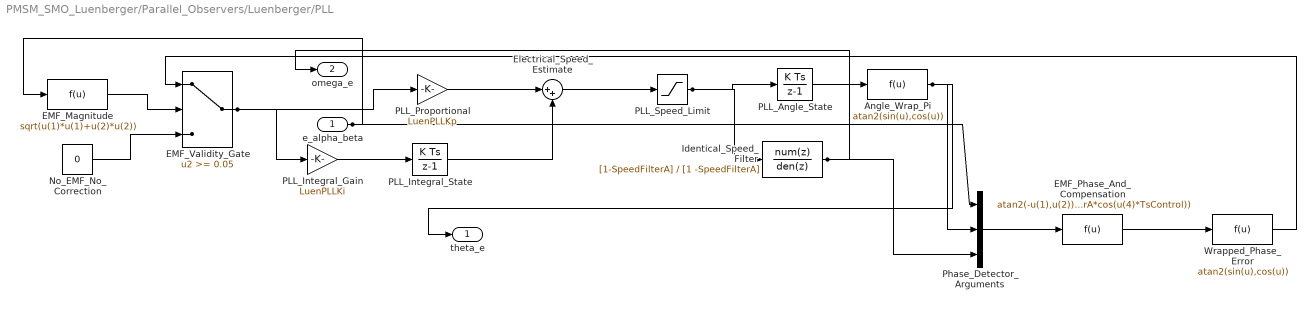
== system PMSM_SMO_Luenberger/Parallel_Observers/Luenberger/PLL ==
  e_alpha_beta : Inport
  Angle_Wrap_Pi : Fcn  Expr=atan2(sin(u),cos(u))
  EMF_Magnitude : Fcn  Expr=sqrt(u(1)*u(1)+u(2)*u(2))
  EMF_Phase_And_Compensation : Fcn  Expr=atan2(-u(1),u(2))-u(3)+atan2(EFilterA*sin(u(4)*TsControl),1-EFilterA*cos(u(4)*TsControl))
  EMF_Validity_Gate : Switch  Threshold=0.05
  Electrical_Speed_Estimate : Sum  Inputs=|++
  Identical_Speed_Filter : DiscreteTransferFcn  Numerator=[1-SpeedFilterA]  Denominator=[1 -SpeedFilterA]  SampleTime=TsControl
  No_EMF_No_Correction : Constant  Value=0
  PLL_Angle_State : DiscreteIntegrator  SampleTime=TsControl  ICPrevOutput=DiscIntNeverNeededParam  ICPrevScaledInput=DiscIntNeverNeededParam
  PLL_Integral_Gain : Gain  Gain=LuenPLLKi
  PLL_Integral_State : DiscreteIntegrator  SampleTime=TsControl  LimitOutput=on  UpperSaturationLimit=1000  LowerSaturationLimit=-1000  ICPrevOutput=DiscIntNeverNeededParam  ICPrevScaledInput=DiscIntNeverNeededParam
  PLL_Proportional : Gain  Gain=LuenPLLKp
  PLL_Speed_Limit : Saturate  UpperLimit=1000  LowerLimit=-1000
  Phase_Detector_Arguments : Mux  Inputs=3
  Wrapped_Phase_Error : Fcn  Expr=atan2(sin(u),cos(u))
  theta_e : Outport
  omega_e : Outport  Port=2
  wires:
  PLL_Angle_State/1 -> Angle_Wrap_Pi/1
  PLL_Speed_Limit/1 -> PLL_Angle_State/1, Identical_Speed_Filter/1
  Electrical_Speed_Estimate/1 -> PLL_Speed_Limit/1
  PLL_Integral_State/1 -> Electrical_Speed_Estimate/2
  PLL_Proportional/1 -> Electrical_Speed_Estimate/1
  PLL_Integral_Gain/1 -> PLL_Integral_State/1
  EMF_Validity_Gate/1 -> PLL_Proportional/1, PLL_Integral_Gain/1
  No_EMF_No_Correction/1 -> EMF_Validity_Gate/3
  EMF_Magnitude/1 -> EMF_Validity_Gate/2
  Wrapped_Phase_Error/1 -> EMF_Validity_Gate/1
  EMF_Phase_And_Compensation/1 -> Wrapped_Phase_Error/1
  Phase_Detector_Arguments/1 -> EMF_Phase_And_Compensation/1
  Identical_Speed_Filter/1 -> omega_e/1, Phase_Detector_Arguments/3
  Angle_Wrap_Pi/1 -> Phase_Detector_Arguments/2, theta_e/1
  e_alpha_beta/1 -> EMF_Magnitude/1, Phase_Detector_Arguments/1

== system PMSM_SMO_Luenberger/Parallel_Observers/SMO/Adaptive_CCF_Bandwidth ==
  Estimated_Omega_radps : Inport
  CCF_Cutoff_Adaptive : MinMax  Function=max  Inputs=2
  CCF_Cutoff_Ratio : Gain  Gain=SmoKe
  CCF_Minimum_Cutoff : Constant  Value=SmoWmin
  Estimated_Speed_Absolute : Abs
  CCF_Bandwidth_radps : Outport
  wires:
  CCF_Cutoff_Adaptive/1 -> CCF_Bandwidth_radps/1
  Estimated_Speed_Absolute/1 -> CCF_Cutoff_Ratio/1
  CCF_Minimum_Cutoff/1 -> CCF_Cutoff_Adaptive/2
  CCF_Cutoff_Ratio/1 -> CCF_Cutoff_Adaptive/1
  Estimated_Omega_radps/1 -> Estimated_Speed_Absolute/1

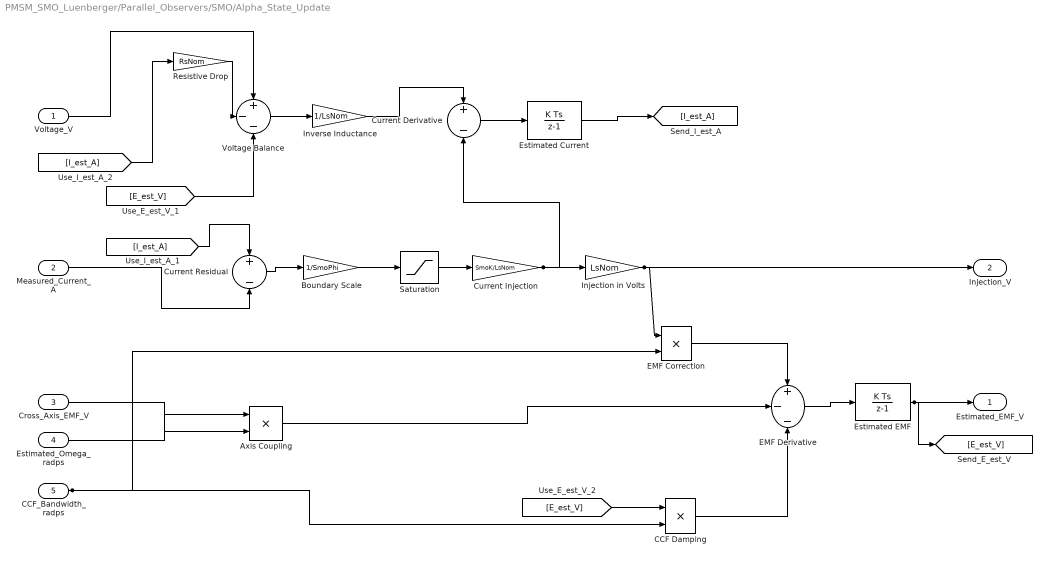
== system PMSM_SMO_Luenberger/Parallel_Observers/SMO/Alpha_State_Update ==
  Voltage_V : Inport
  Measured_Current_A : Inport  Port=2
  Cross_Axis_EMF_V : Inport  Port=3
  Estimated_Omega_radps : Inport  Port=4
  CCF_Bandwidth_radps : Inport  Port=5
  Axis Coupling : Product  Inputs=**
  Boundary Scale : Gain  Gain=1/SmoPhi
  CCF Damping : Product  Inputs=**
  Current Derivative : Sum  Inputs=+-
  Current Injection : Gain  Gain=SmoK/LsNom
  Current Residual : Sum  Inputs=+-
  EMF Correction : Product  Inputs=**
  EMF Derivative : Sum  Inputs=+--
  Estimated Current : DiscreteIntegrator  SampleTime=TsControl  ICPrevOutput=DiscIntNeverNeededParam  ICPrevScaledInput=DiscIntNeverNeededParam
  Estimated EMF : DiscreteIntegrator  SampleTime=TsControl  ICPrevOutput=DiscIntNeverNeededParam  ICPrevScaledInput=DiscIntNeverNeededParam
  Injection in Volts : Gain  Gain=LsNom
  Inverse Inductance : Gain  Gain=1/LsNom
  Resistive Drop : Gain  Gain=RsNom
  Saturation : Saturate  UpperLimit=1  LowerLimit=-1
  Voltage Balance : Sum  Inputs=+--
  Estimated_EMF_V : Outport
  Injection_V : Outport  Port=2
  wires:
  Cross_Axis_EMF_V/1 -> Axis Coupling/2
  CCF_Bandwidth_radps/1 -> EMF Correction/2, CCF Damping/2
  Estimated_Omega_radps/1 -> Axis Coupling/1
  Measured_Current_A/1 -> Current Residual/2
  CCF Damping/1 -> EMF Derivative/3
  Boundary Scale/1 -> Saturation/1
  EMF Derivative/1 -> Estimated EMF/1
  Injection in Volts/1 -> EMF Correction/1, Injection_V/1
  EMF Correction/1 -> EMF Derivative/1
  Saturation/1 -> Current Injection/1
  Axis Coupling/1 -> EMF Derivative/2
  Current Residual/1 -> Boundary Scale/1
  Current Injection/1 -> Current Derivative/2, Injection in Volts/1
  Inverse Inductance/1 -> Current Derivative/1
  [I_est_A] -> Resistive Drop/1
  [I_est_A] -> Current Residual/1
  Current Derivative/1 -> Estimated Current/1
  Resistive Drop/1 -> Voltage Balance/2
  Voltage Balance/1 -> Inverse Inductance/1
  Estimated Current/1 -> [I_est_A]
  Voltage_V/1 -> Voltage Balance/1
  [E_est_V] -> CCF Damping/1
  [E_est_V] -> Voltage Balance/3
  Estimated EMF/1 -> Estimated_EMF_V/1, [E_est_V]

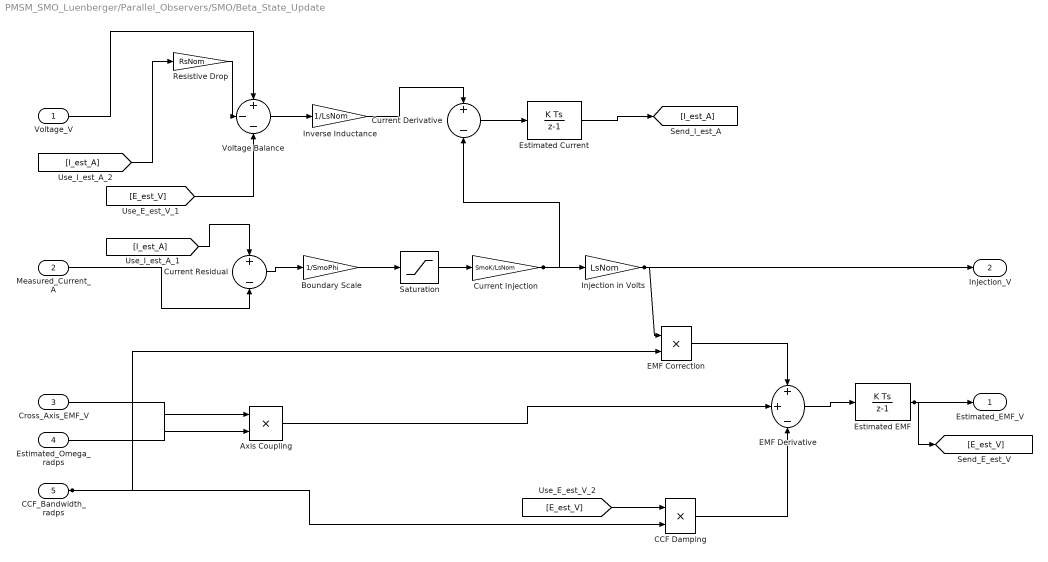
== system PMSM_SMO_Luenberger/Parallel_Observers/SMO/Beta_State_Update ==
  Voltage_V : Inport
  Measured_Current_A : Inport  Port=2
  Cross_Axis_EMF_V : Inport  Port=3
  Estimated_Omega_radps : Inport  Port=4
  CCF_Bandwidth_radps : Inport  Port=5
  Axis Coupling : Product  Inputs=**
  Boundary Scale : Gain  Gain=1/SmoPhi
  CCF Damping : Product  Inputs=**
  Current Derivative : Sum  Inputs=+-
  Current Injection : Gain  Gain=SmoK/LsNom
  Current Residual : Sum  Inputs=+-
  EMF Correction : Product  Inputs=**
  EMF Derivative : Sum  Inputs=++-
  Estimated Current : DiscreteIntegrator  SampleTime=TsControl  ICPrevOutput=DiscIntNeverNeededParam  ICPrevScaledInput=DiscIntNeverNeededParam
  Estimated EMF : DiscreteIntegrator  SampleTime=TsControl  ICPrevOutput=DiscIntNeverNeededParam  ICPrevScaledInput=DiscIntNeverNeededParam
  Injection in Volts : Gain  Gain=LsNom
  Inverse Inductance : Gain  Gain=1/LsNom
  Resistive Drop : Gain  Gain=RsNom
  Saturation : Saturate  UpperLimit=1  LowerLimit=-1
  Voltage Balance : Sum  Inputs=+--
  Estimated_EMF_V : Outport
  Injection_V : Outport  Port=2
  wires:
  Measured_Current_A/1 -> Current Residual/2
  CCF_Bandwidth_radps/1 -> CCF Damping/2, EMF Correction/2
  Estimated_Omega_radps/1 -> Axis Coupling/1
  Boundary Scale/1 -> Saturation/1
  EMF Derivative/1 -> Estimated EMF/1
  CCF Damping/1 -> EMF Derivative/3
  EMF Correction/1 -> EMF Derivative/1
  Saturation/1 -> Current Injection/1
  Cross_Axis_EMF_V/1 -> Axis Coupling/2
  Inverse Inductance/1 -> Current Derivative/1
  Current Residual/1 -> Boundary Scale/1
  Current Injection/1 -> Current Derivative/2, Injection in Volts/1
  Axis Coupling/1 -> EMF Derivative/2
  Injection in Volts/1 -> EMF Correction/1, Injection_V/1
  [I_est_A] -> Resistive Drop/1
  [I_est_A] -> Current Residual/1
  Estimated Current/1 -> [I_est_A]
  Current Derivative/1 -> Estimated Current/1
  Resistive Drop/1 -> Voltage Balance/2
  Voltage Balance/1 -> Inverse Inductance/1
  Voltage_V/1 -> Voltage Balance/1
  [E_est_V] -> CCF Damping/1
  [E_est_V] -> Voltage Balance/3
  Estimated EMF/1 -> Estimated_EMF_V/1, [E_est_V]

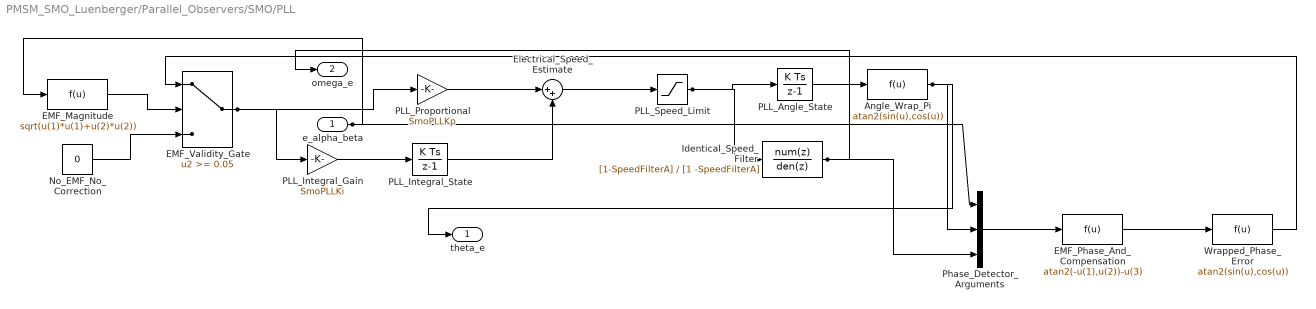
== system PMSM_SMO_Luenberger/Parallel_Observers/SMO/PLL ==
  e_alpha_beta : Inport
  Angle_Wrap_Pi : Fcn  Expr=atan2(sin(u),cos(u))
  EMF_Magnitude : Fcn  Expr=sqrt(u(1)*u(1)+u(2)*u(2))
  EMF_Phase_And_Compensation : Fcn  Expr=atan2(-u(1),u(2))-u(3)
  EMF_Validity_Gate : Switch  Threshold=0.05
  Electrical_Speed_Estimate : Sum  Inputs=|++
  Identical_Speed_Filter : DiscreteTransferFcn  Numerator=[1-SpeedFilterA]  Denominator=[1 -SpeedFilterA]  SampleTime=TsControl
  No_EMF_No_Correction : Constant  Value=0
  PLL_Angle_State : DiscreteIntegrator  SampleTime=TsControl  ICPrevOutput=DiscIntNeverNeededParam  ICPrevScaledInput=DiscIntNeverNeededParam
  PLL_Integral_Gain : Gain  Gain=SmoPLLKi
  PLL_Integral_State : DiscreteIntegrator  SampleTime=TsControl  LimitOutput=on  UpperSaturationLimit=1000  LowerSaturationLimit=-1000  ICPrevOutput=DiscIntNeverNeededParam  ICPrevScaledInput=DiscIntNeverNeededParam
  PLL_Proportional : Gain  Gain=SmoPLLKp
  PLL_Speed_Limit : Saturate  UpperLimit=1000  LowerLimit=-1000
  Phase_Detector_Arguments : Mux  Inputs=3
  Wrapped_Phase_Error : Fcn  Expr=atan2(sin(u),cos(u))
  theta_e : Outport
  omega_e : Outport  Port=2
  wires:
  PLL_Angle_State/1 -> Angle_Wrap_Pi/1
  PLL_Speed_Limit/1 -> PLL_Angle_State/1, Identical_Speed_Filter/1
  Electrical_Speed_Estimate/1 -> PLL_Speed_Limit/1
  PLL_Integral_State/1 -> Electrical_Speed_Estimate/2
  PLL_Proportional/1 -> Electrical_Speed_Estimate/1
  PLL_Integral_Gain/1 -> PLL_Integral_State/1
  EMF_Validity_Gate/1 -> PLL_Proportional/1, PLL_Integral_Gain/1
  No_EMF_No_Correction/1 -> EMF_Validity_Gate/3
  EMF_Magnitude/1 -> EMF_Validity_Gate/2
  Wrapped_Phase_Error/1 -> EMF_Validity_Gate/1
  EMF_Phase_And_Compensation/1 -> Wrapped_Phase_Error/1
  Phase_Detector_Arguments/1 -> EMF_Phase_And_Compensation/1
  Identical_Speed_Filter/1 -> omega_e/1, Phase_Detector_Arguments/3
  Angle_Wrap_Pi/1 -> Phase_Detector_Arguments/2, theta_e/1
  e_alpha_beta/1 -> EMF_Magnitude/1, Phase_Detector_Arguments/1
